simulink model "system_simulation_training_creator"  (R2026b)
settings: Solver=FixedStepAuto  StopTime=60  FixedStep=Ts
undefined symbols (not defined in the file or in its folder): Ts
settings Model: Creator=Max  LastModifiedBy=ctamboise

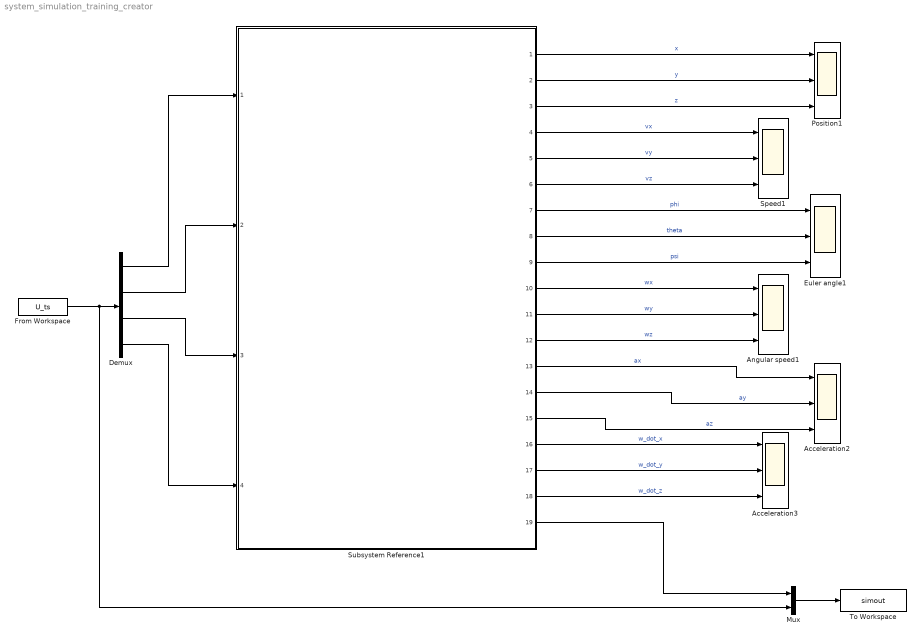
== system system_simulation_training_creator ==
  Acceleration2 : Scope  NumInputPorts=3
      settings: ActiveDisplayYMinimum=-13.59687263842237  ActiveDisplayYMaximum=10.248111830599871  DataLoggingVariableName=ScopeData7
  Acceleration3 : Scope  NumInputPorts=3
      settings: ActiveDisplayYMinimum=-40.918121722117149  ActiveDisplayYMaximum=44.001627281329164  DataLoggingVariableName=ScopeData8
  Angular speed1 : Scope  NumInputPorts=3
      settings: ActiveDisplayYMinimum=-1  ActiveDisplayYMaximum=1  DataLoggingVariableName=ScopeData9
  Demux : Demux
  Euler angle1 : Scope  NumInputPorts=3
      settings: ActiveDisplayYMinimum=-1695.66598  ActiveDisplayYMaximum=1344.64163  DataLoggingVariableName=ScopeData10
  From Workspace : FromWorkspace  VariableName=U_ts  SampleTime=Ts  Interpolate=off  OutputAfterFinalValue=Holding final value
  Mux : Mux  Inputs=2
  Position1 : Scope  NumInputPorts=3
      settings: ActiveDisplayYMinimum=-7.0564531577369323  ActiveDisplayYMaximum=0.78348256156553819  DataLoggingVariableName=ScopeData11
  Speed1 : Scope  NumInputPorts=3
      settings: ActiveDisplayYMinimum=-2.0291599170695513  ActiveDisplayYMaximum=0.93228871088825449  DataLoggingVariableName=ScopeData12
  Subsystem Reference1 : Subsystem  ReferencedSubsystem=UAV_model
  To Workspace : ToWorkspace  VariableName=simout  SaveFormat=Structure With Time  SampleTime=Ts
  wires:
  Subsystem Reference1/18 -> Acceleration3/3  "w_dot_z"
  Subsystem Reference1/17 -> Acceleration3/2  "w_dot_y"
  Subsystem Reference1/7 -> Euler angle1/1  "phi"
  Subsystem Reference1/5 -> Speed1/2  "vy"
  Subsystem Reference1/3 -> Position1/3  "z"
  Subsystem Reference1/6 -> Speed1/3  "vz"
  Subsystem Reference1/19 -> Mux/1
  Subsystem Reference1/4 -> Speed1/1  "vx"
  Subsystem Reference1/9 -> Euler angle1/3  "psi"
  Subsystem Reference1/16 -> Acceleration3/1  "w_dot_x"
  Subsystem Reference1/12 -> Angular speed1/3  "wz"
  Subsystem Reference1/8 -> Euler angle1/2  "theta"
  Subsystem Reference1/15 -> Acceleration2/3  "az"
  Subsystem Reference1/11 -> Angular speed1/2  "wy"
  Subsystem Reference1/2 -> Position1/2  "y"
  Subsystem Reference1/10 -> Angular speed1/1  "wx"
  Subsystem Reference1/14 -> Acceleration2/2  "ay"
  Subsystem Reference1/1 -> Position1/1  "x"
  Subsystem Reference1/13 -> Acceleration2/1  "ax"
  Demux/4 -> Subsystem Reference1/4
  Demux/1 -> Subsystem Reference1/1
  Demux/2 -> Subsystem Reference1/2
  Demux/3 -> Subsystem Reference1/3
  From Workspace/1 -> Mux/2, Demux/1
  Mux/1 -> To Workspace/1
